simulink model "vita_sys_004"  (R2025b)
settings: Solver=VariableStepAuto  StartTime=0.0  StopTime=30  RelTol=1e-3
undefined symbols (not defined in the file): driving
libraries: drivingscenarioandsensors x2
settings Model: Creator=ADMIIN  LastModifiedBy=ADMIIN

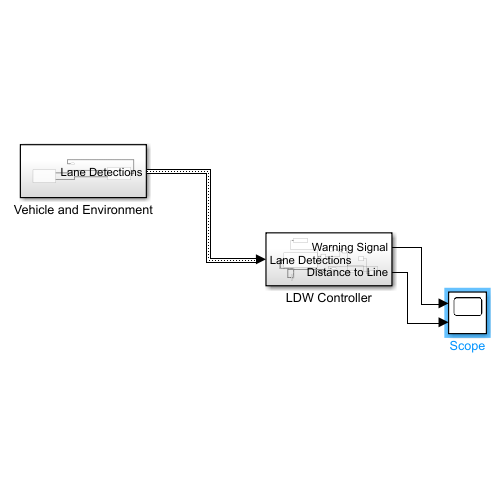
[thumbnail: Simulink's stored preview of the top-level diagram]
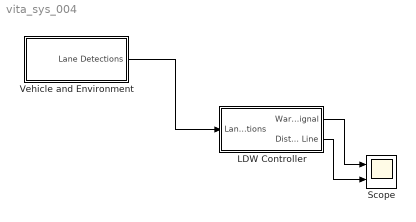
== system vita_sys_004 ==
  LDW Controller : Subsystem
  Scope : Scope  NumInputPorts=2
      settings: ActiveDisplayYMinimum=-2.6300649792144926  ActiveDisplayYMaximum=1.5266943604501892
  Vehicle and Environment : Subsystem
  wires:
  LDW Controller/1(Warning Signal) -> Scope/1
  Vehicle and Environment/1(Lane Detections) -> LDW Controller/1(Lane Detections)
  LDW Controller/2(Distance to Line) -> Scope/2

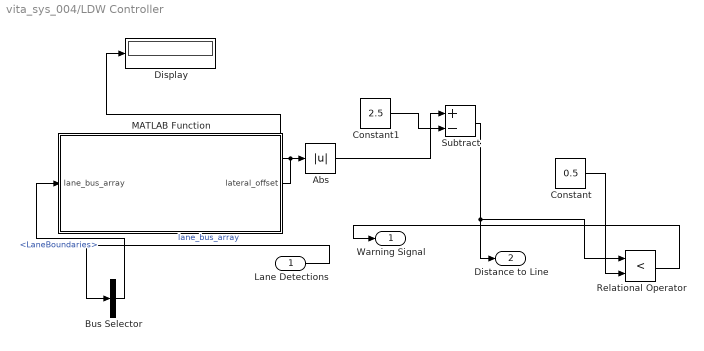
== system vita_sys_004/LDW Controller ==
  Lane Detections : Inport
  Abs : Abs  SaturateOnIntegerOverflow=off
  Bus Selector : BusSelector  OutputSignals=LaneBoundaries
  Constant : Constant  Value=0.5
  Constant1 : Constant  Value=2.5
  Display : Display
  MATLAB Function : MATLAB Function  TreatAsAtomicUnit=on
  Relational Operator : RelationalOperator  Operator=<  OutDataTypeStr=boolean  RndMeth=Simplest  InputSameDT=off
  Subtract : Sum  Inputs=+-
  Warning Signal : Outport
  Distance to Line : Outport  Port=2
  wires:
  Subtract/1 -> Relational Operator/1, Distance to Line/1
  Constant/1 -> Relational Operator/2
  Relational Operator/1 -> Warning Signal/1
  MATLAB Function/1(lateral_offset) -> Display/1, Abs/1
  Lane Detections/1 -> Bus Selector/1  "lane_bus_array"
  Bus Selector/1 -> MATLAB Function/1(lane_bus_array)  "<LaneBoundaries>"
  Constant1/1 -> Subtract/2
  Abs/1 -> Subtract/1

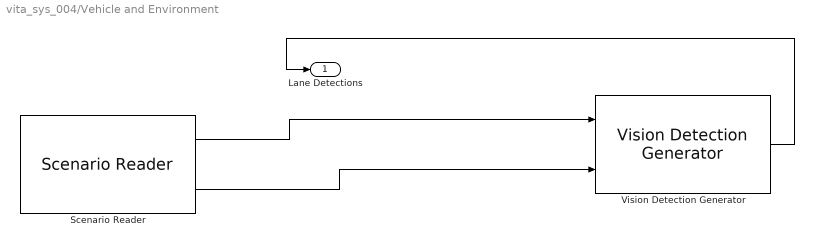
== system vita_sys_004/Vehicle and Environment ==
  Scenario Reader : drivingscenarioandsensors/Scenario Reader  ScenarioSource=From file  ScenarioFileName=E:\tata\ldw_scenario.mat  ScenarioVariableName=scenario  OutputCoordinateSystem=Vehicle coordinates  EgoVehicleSource=Scenario  EgoVehicleActorID=1  OrientVehiclesOnRoad=off  OutputEgoVehiclePose=off  OutputEgoVehicleState=off  SampleTime=0.1  LaneBoundaryOutput=Ego vehicle lane boundaries  LaneBoundaryDistance=0:0.5:9.5  LaneBoundaryLocation=Center of lane markings  BusNameSource=Auto  BusName=BusActors  BusNumActorsSource=Scenario  BusNumActors=100  BusName2Source=Auto  BusName2=BusLaneBoundaries  BusNumLaneBoundariesSource=Scenario  BusNumLaneBoundaries=10  BusName3Source=Auto  BusName3=BusEgoActor  BusName4Source=Auto  BusName4=BusEgoState  ShowCoordinateLabels=on  SimulateUsing=Interpreted execution
  Vision Detection Generator : drivingscenarioandsensors/Vision Detection Generator  SensorIndex=1  DetectorOutput=Lanes with occlusion  UpdateInterval=0.1  LaneUpdateInterval=0.1  SensorLocation=[ 1.9, 0 ]  Height=1.1  Yaw=0  Pitch=1  Roll=0  BusNameSource=Auto  BusName=BusObjectDetections  BusName2Source=Auto  BusName2=BusLaneDetections  MaxNumDetectionsSource=Property  MaxNumDetections=50  MaxNumLanesSource=Property  MaxNumLanes=30  DetectionCoordinates=Ego Cartesian  SimulateUsing=Interpreted execution  MaxRange=150  BoundingBoxAccuracy=5  ProcessNoiseIntensity=5  MaxSpeed=100  MaxAllowedOcclusion=0.5  MinObjectImageSize=[ 15, 15 ]  DetectionProbability=0.9  FalsePositivesPerImage=0.1  MinLaneImageSize=[ 20, 3 ]  LaneBoundaryAccuracy=3  HasNoise=on  InitialSeedSource=Repeatable  InitialSeed=0  UsedSeed=driving.internal.SimulinkUtilities.seedManager(gcb)  ActorProfilesSource=From Scenario Reader block  ActorProfilesParameters=driving.internal.ActorProfilesParameters  ActorProfilesExpression=struct( 'ClassID', 0, 'Length', 4.7, 'Width', 1.8, 'Height', 1.4, 'OriginOffset', [ -1.35, 0, 0 ] )  Intrinsics=driving.internal.cameraIntrinsics
  Lane Detections : Outport
  wires:
  Vision Detection Generator/1 -> Lane Detections/1
  Scenario Reader/1 -> Vision Detection Generator/1
  Scenario Reader/2 -> Vision Detection Generator/2

== matlab function vita_sys_004/LDW Controller/MATLAB Function ==
  data: lane_bus_array input; lateral_offset output
function lateral_offset = get_first_lane_offset(lane_bus_array)
% This function takes the array of lane boundary buses and returns the
% LateralOffset of the first detected lane.
% Default value if no lanes are detected
 lateral_offset = 0;
% Check if the vision sensor detected at least one lane
if ~isempty(lane_bus_array)
% Get the LateralOffset from the first lane in the array
 lateral_offset = lane_bus_array(1).LateralOffset;
end
end
